simulink model "mission_LQ"  (R2025b)
settings: Solver=VariableStepAuto  StartTime=0.0  StopTime=50  RelTol=1e-3
values from neighbouring files (symbols this model uses):
  h_v = 0    [parametres_mission_LQ.m]
  v_v = 0.3    [parametres_mission_LQ.m]
  x_v0 = 1    [parametres_mission_LQ.m]
undefined symbols (not defined in the file or in its folder): DiscIntNeverNeededParam, Kd, Kd_psi, Kd_theta, Kd_x, Ki, Ki_psi, Ki_theta, Kp, Kp_psi, Kp_theta, Kp_x, theta_max, V_max
settings Model: Creator=anoua  LastModifiedBy=anoua

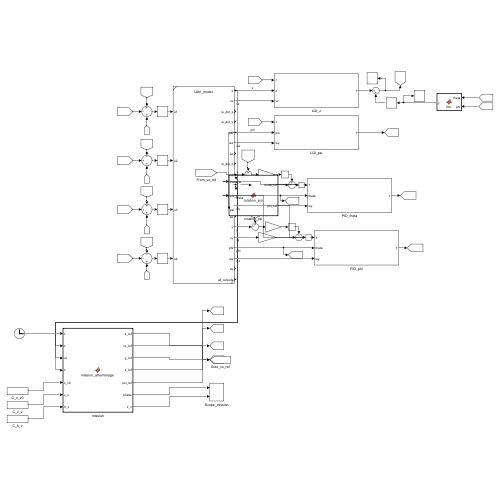
[thumbnail: Simulink's stored preview of the top-level diagram]
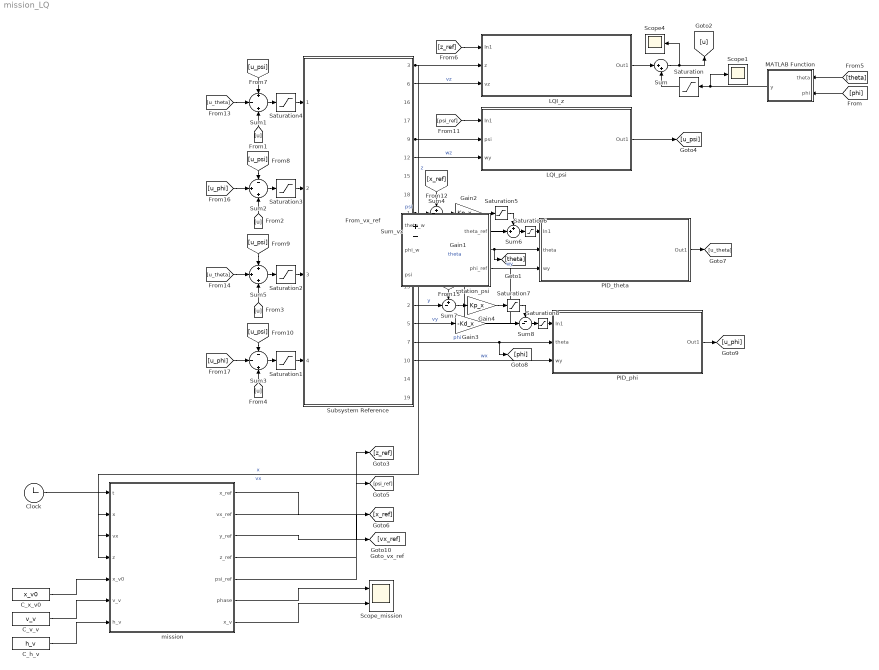
== system mission_LQ ==
  C_h_v : Constant  Value=h_v
  C_v_v : Constant  Value=v_v
  C_x_v0 : Constant  Value=x_v0
  Clock : Clock
  Gain1 : Gain  Gain=Kd_x
  Gain2 : Gain  Gain=Kp_x
  Gain3 : Gain  Gain=-Kd_x
  Gain4 : Gain  Gain=Kp_x
  LQI_psi : Subsystem
  LQI_z : Subsystem
  MATLAB Function : MATLAB Function  TreatAsAtomicUnit=on
  PID_phi : Subsystem
  PID_theta : Subsystem
  Saturation : Saturate  UpperLimit=0.41  LowerLimit=0.35
  Saturation{1..4} (4 alike) : Saturate  UpperLimit=1  LowerLimit=-1
  Saturation5 : Saturate  UpperLimit=V_max*Kd_x  LowerLimit=-V_max*Kd_x
  Saturation6 : Saturate  UpperLimit=theta_max  LowerLimit=-theta_max
  Saturation7 : Saturate  UpperLimit=V_max*Kd_x  LowerLimit=-V_max*Kd_x
  Saturation8 : Saturate  UpperLimit=theta_max  LowerLimit=-theta_max
  Scope1 : Scope
      settings: ActiveDisplayYMinimum=0.38999944331549796  ActiveDisplayYMaximum=0.39000055810737394
  Scope4 : Scope
      settings: ActiveDisplayYMinimum=-4.4218137268268194  ActiveDisplayYMaximum=39.350730126019634  DataLoggingVariableName=ScopeData4
  Scope_mission : Scope  NumInputPorts=2
  Subsystem Reference : Subsystem  ReferencedSubsystem=UAV_model
      settings: PortSchema="{\"entries\":[{\"content\":{\"sides\":[{\"content\":{\"connectorIds\":[\"In1\",\"In2\",\"In3\",\"In4\"]},\"type\":\"ConnectorPlacement.EquallySpacedRectSide\",\"uuid\":\"01aa2ccd-8bb1-4ec5-b7fa-b8cd375824c1\"},{\"content\":{\"connectorIds\":[\"Out3\",\"Out6\",\"Out16\",\"Out17\",\"Out9\",\"Out12\",\"Out15\",\"Out18\",\"Out1\",\"Out4\",\"Out8\",\"Out11\",\"Out13\",\"Out2\",\"Out5\",\"Out7\",\"Out10\",\"Out14\",\"Out19\"],\"side\":\"RIGHT\"},\"type\":\"ConnectorPlacement.EquallySpacedRectSide\",\"uuid\":\"5e4cf163-674c-4c62-8457-5b263a3040bc\"},{\"content\":{\"side\":\"TOP\"},\"type\":\"ConnectorPlacement.EquallySpacedRectSide\",\"uuid\":\"9ea84534-8679-4237-9c2b-2b22f3a10628\"}]},\"type\":\"ConnectorPlacement.EquallySpacedConnector\",\"uuid\":\"5e8d904e-05ef-4f02-905a-9e7f0437b2a0\"}],\"packageUris\":[\"http://schema.mathworks.com/mf0/Connector/R2020b\"],\"version\":\"1.0\"}"
  Sum : Sum  Inputs=|++
  Sum1 : Sum  Inputs=+|-|+
  Sum2 : Sum  Inputs=-|+|+
  Sum3 : Sum  Inputs=-|-|+
  Sum4 : Sum  Inputs=+-|
  Sum5 : Sum  Inputs=+|+|+
  Sum6 : Sum  Inputs=++|
  Sum7 : Sum  Inputs=+-|
  Sum8 : Sum  Inputs=--|
  Sum_vx : Sum  Inputs=+-
  mission : MATLAB Function  TreatAsAtomicUnit=on
  rotation_psi : MATLAB Function  TreatAsAtomicUnit=on
  wires:
  Saturation/1 -> Sum/2
  Sum/1 -> Scope4/1, [u]
  LQI_z/1(Out1) -> Sum/1
  Subsystem Reference/3 -> LQI_z/2(z), mission/4(z)  "z"
  Subsystem Reference/6 -> LQI_z/3(vz)  "vz"
  [theta] -> MATLAB Function/1(theta)
  [phi] -> MATLAB Function/2(phi)
  Sum1/1 -> Saturation4/1
  MATLAB Function/1(y) -> Scope1/1, Saturation/1
  [z_ref] -> LQI_z/1(In1)
  Subsystem Reference/9 -> LQI_psi/2(psi), rotation_psi/3(psi)  "psi"
  LQI_psi/1(Out1) -> [u_psi]
  [u] -> Sum1/3
  [u_psi] -> Sum1/1
  [u] -> Sum2/3
  [u] -> Sum5/3
  [u] -> Sum3/3
  [u_psi] -> Sum2/1
  [u_psi] -> Sum5/1
  [u_psi] -> Sum3/1
  [psi_ref] -> LQI_psi/1(In1)
  Subsystem Reference/1 -> Sum4/2, mission/2(x)  "x"
  [x_ref] -> Sum4/1
  Sum4/1 -> Gain2/1
  Subsystem Reference/4 -> mission/3(vx), Sum_vx/2  "vx"
  Gain2/1 -> Saturation5/1
  Gain1/1 -> Sum6/2
  Saturation5/1 -> Sum6/1
  Saturation6/1 -> PID_theta/1(In1)
  Subsystem Reference/8 -> [theta], PID_theta/2(theta)  "theta"
  Subsystem Reference/12 -> LQI_psi/3(wy)  "wz"
  Subsystem Reference/11 -> PID_theta/3(wy)  "wy"
  PID_theta/1(Out1) -> [u_theta]
  [u_theta] -> Sum1/2
  [u_theta] -> Sum5/2
  [y_ref] -> Sum7/1
  Saturation8/1 -> PID_phi/1(In1)
  PID_phi/1(Out1) -> [u_phi]
  Sum7/1 -> Gain4/1
  Saturation7/1 -> Sum8/1
  Gain4/1 -> Saturation7/1
  Gain3/1 -> Sum8/2
  Subsystem Reference/2 -> Sum7/2  "y"
  Subsystem Reference/5 -> Gain3/1  "vy"
  Subsystem Reference/7 -> [phi], PID_phi/2(theta)  "phi"
  Subsystem Reference/10 -> PID_phi/3(wy)  "wx"
  [u_phi] -> Sum2/2
  [u_phi] -> Sum3/2
  Saturation4/1 -> Subsystem Reference/1
  Sum2/1 -> Saturation3/1
  Saturation3/1 -> Subsystem Reference/2
  Sum5/1 -> Saturation2/1
  Saturation2/1 -> Subsystem Reference/3
  Sum3/1 -> Saturation1/1
  Saturation1/1 -> Subsystem Reference/4
  Clock/1 -> mission/1(t)
  C_x_v0/1 -> mission/5(x_v0)
  C_v_v/1 -> mission/6(v_v)
  C_h_v/1 -> mission/7(h_v)
  mission/1(x_ref) -> [x_ref]
  mission/3(y_ref) -> [y_ref]
  mission/4(z_ref) -> [z_ref]
  mission/5(psi_ref) -> [psi_ref]
  mission/2(vx_ref) -> [vx_ref]
  mission/6(phase) -> Scope_mission/1
  mission/7(x_v) -> Scope_mission/2
  [vx_ref] -> Sum_vx/1
  Sum_vx/1 -> Gain1/1
  Sum6/1 -> rotation_psi/1(theta_w)
  Sum8/1 -> rotation_psi/2(phi_w)
  rotation_psi/1(theta_ref) -> Saturation6/1
  rotation_psi/2(phi_ref) -> Saturation8/1

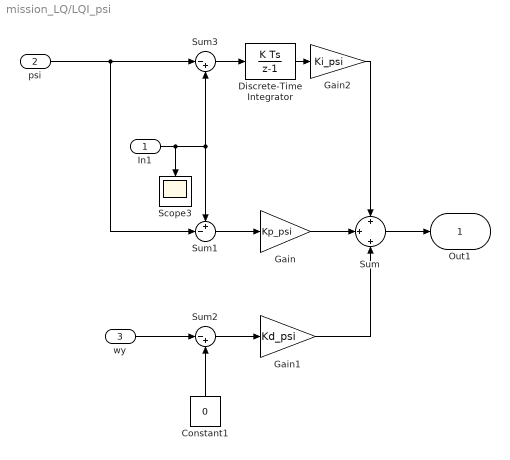
== system mission_LQ/LQI_psi ==
  In1 : Inport
  psi : Inport  Port=2
  wy : Inport  Port=3
  Constant1 : Constant  Value=0
  Discrete-Time Integrator : DiscreteIntegrator  SampleTime=-1  LimitOutput=on  UpperSaturationLimit=1/Ki_psi  LowerSaturationLimit=-1/Ki_psi  ICPrevOutput=DiscIntNeverNeededParam  ICPrevScaledInput=DiscIntNeverNeededParam
  Gain : Gain  Gain=Kp_psi
  Gain1 : Gain  Gain=Kd_psi
  Gain2 : Gain  Gain=Ki_psi
  Scope3 : Scope
      settings: ActiveDisplayYMinimum=-0.53484809981403014  ActiveDisplayYMaximum=1.6271171549271228  DataLoggingVariableName=ScopeData3
  Sum : Sum  Inputs=+|+|+
  Sum1 : Sum  Inputs=+-|
  Sum2 : Sum  Inputs=|-+
  Sum3 : Sum  Inputs=|-+
  Out1 : Outport
  wires:
  Gain2/1 -> Sum/1
  Gain/1 -> Sum/2
  Sum2/1 -> Gain1/1
  Gain1/1 -> Sum/3
  In1/1 -> Sum3/2, Sum1/1, Scope3/1
  Sum1/1 -> Gain/1
  Discrete-Time Integrator/1 -> Gain2/1
  Constant1/1 -> Sum2/2
  Sum3/1 -> Discrete-Time Integrator/1
  Sum/1 -> Out1/1
  psi/1 -> Sum1/2, Sum3/1
  wy/1 -> Sum2/1

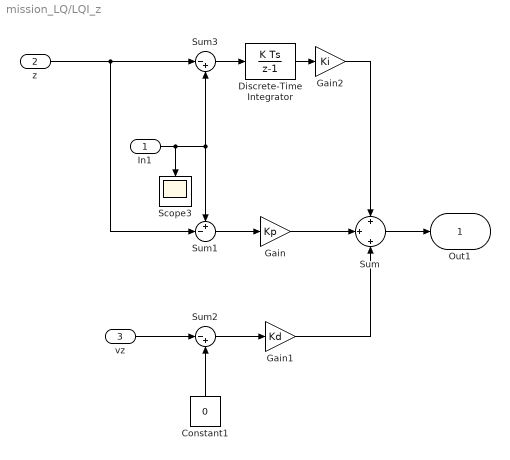
== system mission_LQ/LQI_z ==
  In1 : Inport
  z : Inport  Port=2
  vz : Inport  Port=3
  Constant1 : Constant  Value=0
  Discrete-Time Integrator : DiscreteIntegrator  SampleTime=-1  LimitOutput=on  UpperSaturationLimit=1/Ki  LowerSaturationLimit=-1/Ki  ICPrevOutput=DiscIntNeverNeededParam  ICPrevScaledInput=DiscIntNeverNeededParam
  Gain : Gain  Gain=Kp
  Gain1 : Gain  Gain=Kd
  Gain2 : Gain  Gain=Ki
  Scope3 : Scope
      settings: ActiveDisplayYMinimum=-0.53484809981403014  ActiveDisplayYMaximum=1.6271171549271228  DataLoggingVariableName=ScopeData3
  Sum : Sum  Inputs=+|+|+
  Sum1 : Sum  Inputs=+-|
  Sum2 : Sum  Inputs=|-+
  Sum3 : Sum  Inputs=|-+
  Out1 : Outport
  wires:
  Gain2/1 -> Sum/1
  Gain/1 -> Sum/2
  Sum2/1 -> Gain1/1
  Gain1/1 -> Sum/3
  In1/1 -> Sum3/2, Sum1/1, Scope3/1
  Sum1/1 -> Gain/1
  Discrete-Time Integrator/1 -> Gain2/1
  Constant1/1 -> Sum2/2
  Sum3/1 -> Discrete-Time Integrator/1
  Sum/1 -> Out1/1
  z/1 -> Sum1/2, Sum3/1
  vz/1 -> Sum2/1

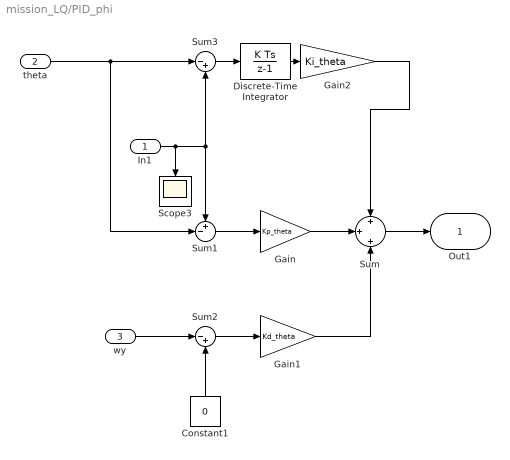
== system mission_LQ/PID_phi ==
  In1 : Inport
  theta : Inport  Port=2
  wy : Inport  Port=3
  Constant1 : Constant  Value=0
  Discrete-Time Integrator : DiscreteIntegrator  SampleTime=-1  LimitOutput=on  UpperSaturationLimit=1/Ki_theta  LowerSaturationLimit=-1/Ki_theta  ICPrevOutput=DiscIntNeverNeededParam  ICPrevScaledInput=DiscIntNeverNeededParam
  Gain : Gain  Gain=Kp_theta
  Gain1 : Gain  Gain=Kd_theta
  Gain2 : Gain  Gain=Ki_theta
  Scope3 : Scope
      settings: ActiveDisplayYMinimum=-0.53484809981403014  ActiveDisplayYMaximum=1.6271171549271228  DataLoggingVariableName=ScopeData3
  Sum : Sum  Inputs=+|+|+
  Sum1 : Sum  Inputs=+-|
  Sum2 : Sum  Inputs=|-+
  Sum3 : Sum  Inputs=|-+
  Out1 : Outport
  wires:
  Gain2/1 -> Sum/1
  Gain/1 -> Sum/2
  Sum2/1 -> Gain1/1
  Gain1/1 -> Sum/3
  In1/1 -> Sum3/2, Sum1/1, Scope3/1
  Sum1/1 -> Gain/1
  Discrete-Time Integrator/1 -> Gain2/1
  Constant1/1 -> Sum2/2
  Sum3/1 -> Discrete-Time Integrator/1
  Sum/1 -> Out1/1
  theta/1 -> Sum1/2, Sum3/1
  wy/1 -> Sum2/1

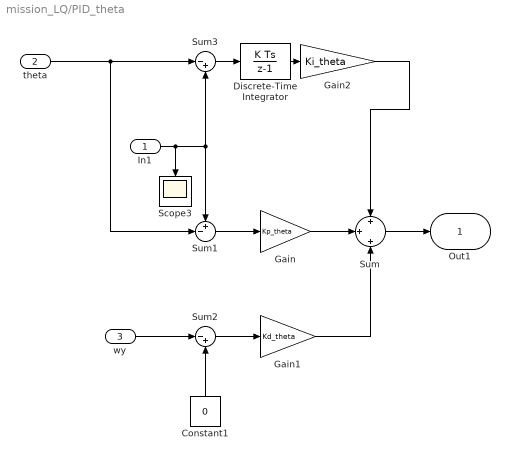
== system mission_LQ/PID_theta ==
  In1 : Inport
  theta : Inport  Port=2
  wy : Inport  Port=3
  Constant1 : Constant  Value=0
  Discrete-Time Integrator : DiscreteIntegrator  SampleTime=-1  LimitOutput=on  UpperSaturationLimit=1/Ki_theta  LowerSaturationLimit=-1/Ki_theta  ICPrevOutput=DiscIntNeverNeededParam  ICPrevScaledInput=DiscIntNeverNeededParam
  Gain : Gain  Gain=Kp_theta
  Gain1 : Gain  Gain=Kd_theta
  Gain2 : Gain  Gain=Ki_theta
  Scope3 : Scope
      settings: ActiveDisplayYMinimum=-0.53484809981403014  ActiveDisplayYMaximum=1.6271171549271228  DataLoggingVariableName=ScopeData3
  Sum : Sum  Inputs=+|+|+
  Sum1 : Sum  Inputs=+-|
  Sum2 : Sum  Inputs=|-+
  Sum3 : Sum  Inputs=|-+
  Out1 : Outport
  wires:
  Gain2/1 -> Sum/1
  Gain/1 -> Sum/2
  Sum2/1 -> Gain1/1
  Gain1/1 -> Sum/3
  In1/1 -> Sum3/2, Sum1/1, Scope3/1
  Sum1/1 -> Gain/1
  Discrete-Time Integrator/1 -> Gain2/1
  Constant1/1 -> Sum2/2
  Sum3/1 -> Discrete-Time Integrator/1
  Sum/1 -> Out1/1
  theta/1 -> Sum1/2, Sum3/1
  wy/1 -> Sum2/1

== matlab function mission_LQ/rotation_psi ==
  data: theta_w input; theta_ref output; phi_w input; psi input; phi_ref output
function [theta_ref, phi_ref] = rotation_psi(theta_w, phi_w, psi)
% theta_w : commande pour avancer en x monde ; phi_w : commande pour y monde (signe deja inverse)
c_x = theta_w;  c_y = -phi_w;            % acceleration souhaitee dans le repere monde
c_xb =  cos(psi)*c_x + sin(psi)*c_y;     % projection dans le repere du drone
c_yb = -sin(psi)*c_x + cos(psi)*c_y;
theta_ref = c_xb;  phi_ref = -c_yb;      % +theta -> +x_b ; +phi -> -y_b
end

== matlab function mission_LQ/mission ==
  settings: updateMethod=DISCRETE  sampleTime=0.05
  data: t input; x_ref output; x input; vx input; z input; x_v0 input; v_v input; h_v input; vx_ref output; y_ref output; z_ref output; psi_ref output; phase output; x_v output
function [x_ref, vx_ref, y_ref, z_ref, psi_ref, phase, x_v] = mission_atterrissage(t, x, vx, z, x_v0, v_v, h_v)
% Séquenceur de mission : décollage -> scan 360° -> poursuite -> descente -> posé
% Appelé toutes les 0.05 s (pas d'échantillonnage du bloc).
persistent ph d0 t3 t_ok t4
if isempty(ph), ph = 1; d0 = 0; t3 = 0; t_ok = 0; t4 = 0; end

Z_VOL    = 0.5;   % altitude de vol (m)
T_MONTEE = 5;     % durée de la rampe de décollage (s)
T_SCAN   = 10;    % durée du tour complet (s) -> 0.63 rad/s
T_APP    = 3;     % constante de temps de l'approche (s)
V_DESC   = 0.1;   % vitesse de descente (m/s)
TOL_X    = 0.05;  % tolérance d'alignement en position (m)
TOL_V    = 0.05;  % tolérance d'alignement en vitesse (m/s)

x_v = x_v0 + v_v * t;            % voiture : mouvement rectiligne uniforme selon x
x_ref = 0; vx_ref = 0; y_ref = 0;
z_ref = Z_VOL * min(t / T_MONTEE, 1);
psi_ref = 0;

% --- transitions et consignes
if ph == 1 && t >= T_MONTEE, ph = 2; end
if ph >= 2
    psi_ref = 2 * pi * min((t - T_MONTEE) / T_SCAN, 1);   % vitesse constante puis maintien à 2*pi
end
if ph == 2 && t >= T_MONTEE + T_SCAN
    ph = 3; t3 = t; d0 = x_v - x;                          % écart au début de la poursuite
end
if ph >= 3
    s = (t - t3) / T_APP;
    e = exp(-s);
    x_ref  = x_v - d0 * (1 + s) * e;                       % approche critique : part du drone, vitesse relative initiale nulle
    vx_ref = v_v + d0 / T_APP * s * e;
    z_ref  = Z_VOL;
end
if ph == 3
    if abs(x - x_v) < TOL_X && abs(vx - v_v) < TOL_V, t_ok = t_ok + 0.05; else, t_ok = 0; end
    if t_ok >= 1, ph = 4; t4 = t; end
end
if ph >= 4
    z_ref = max(Z_VOL - V_DESC * (t - t4), h_v);
    if ph == 4 && z - h_v < 0.02, ph = 5; end
end
phase = ph;
end

== matlab function mission_LQ/MATLAB Function ==
  data: theta input; y output; phi input
function y = fcn(theta,phi)

y= 0.39/(cos(theta)*cos(phi));
